simulink model "torque_vectoring_sim"  (R2022a)
settings: Solver=FixedStepAuto  StartTime=0.0  StopTime=5  FixedStep=0.01  RelTol=1e-3
undefined symbols (not defined in the file): DiscIntNeverNeededParam
libraries: simulink_extras x2, simulink x1
(part 1 of 2)
settings Model: Creator=mdrew  LastModifiedBy=mdrew

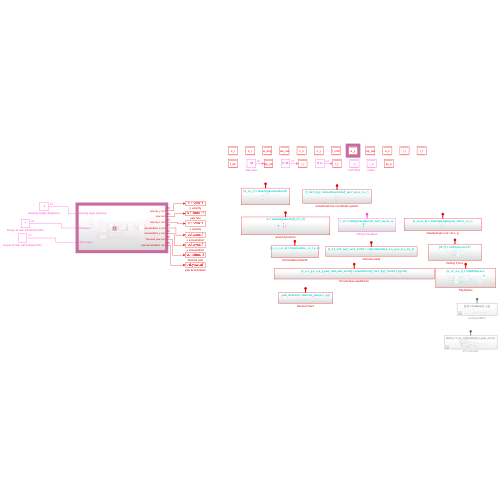
[thumbnail: Simulink's stored preview of the top-level diagram]
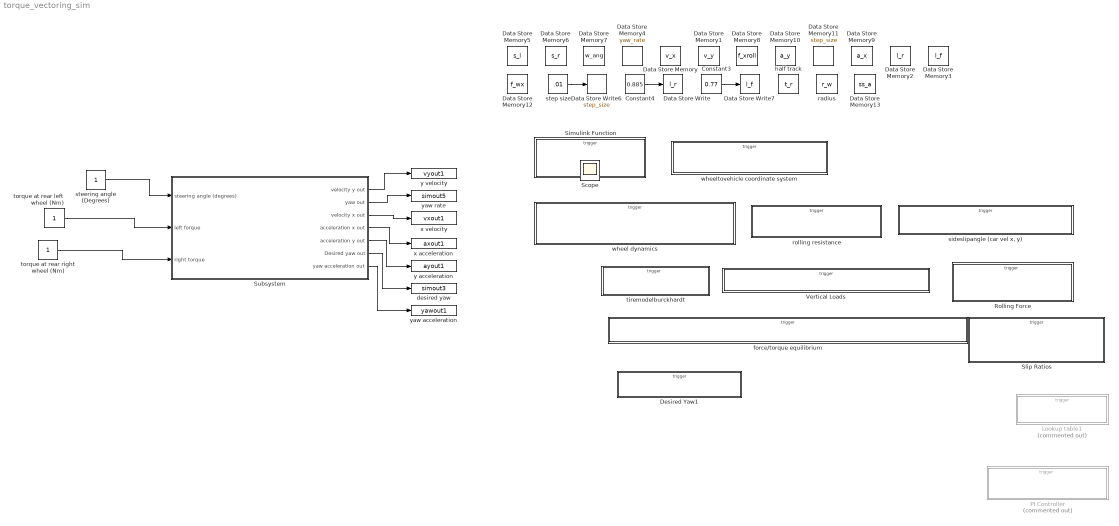
== system torque_vectoring_sim ==
  Constant3 : Constant  Value=0.77
  Constant4 : Constant  Value=0.885
  Data Store Memory : DataStoreMemory  DataStoreName=v_x  WriteAfterWriteMsg=warning  InitialValue=0.1  ShowAdditionalParam=off  OutMin=-10  OutMax=20
  Data Store Memory1 : DataStoreMemory  DataStoreName=v_y  WriteAfterWriteMsg=warning  InitialValue=0.0001  ShowAdditionalParam=off
  Data Store Memory10 : DataStoreMemory  DataStoreName=a_y  WriteAfterWriteMsg=warning  ShowAdditionalParam=off
  Data Store Memory11 : DataStoreMemory  DataStoreName=step_size  WriteAfterWriteMsg=warning  InitialValue=0.01  ShowAdditionalParam=off
  Data Store Memory12 : DataStoreMemory  DataStoreName=f_wx  WriteAfterWriteMsg=warning  InitialValue=[0.1, 0.1, 0.1, 0.1]  ShowAdditionalParam=off
  Data Store Memory13 : DataStoreMemory  DataStoreName=ss_a  WriteAfterWriteMsg=warning  InitialValue=[0, 0, 0, 0]  ShowAdditionalParam=off
  Data Store Memory2 : DataStoreMemory  DataStoreName=l_r  WriteAfterWriteMsg=warning  ShowAdditionalParam=off
  Data Store Memory3 : DataStoreMemory  DataStoreName=l_f  WriteAfterWriteMsg=warning  ShowAdditionalParam=off
  Data Store Memory4 : DataStoreMemory  DataStoreName=yaw_rate  WriteAfterWriteMsg=warning  InitialValue=0.001  ShowAdditionalParam=off
  Data Store Memory5 : DataStoreMemory  DataStoreName=s_l  WriteAfterWriteMsg=warning  ShowAdditionalParam=off
  Data Store Memory6 : DataStoreMemory  DataStoreName=s_r  WriteAfterWriteMsg=warning  ShowAdditionalParam=off
  Data Store Memory7 : DataStoreMemory  DataStoreName=w_ang  WriteAfterWriteMsg=warning  ShowAdditionalParam=off  Dimensions=4
  Data Store Memory8 : DataStoreMemory  DataStoreName=f_xroll  WriteAfterWriteMsg=warning  InitialValue=[.01, .01, .01, .01]  ShowAdditionalParam=off  Dimensions=4
  Data Store Memory9 : DataStoreMemory  DataStoreName=a_x  WriteAfterWriteMsg=warning  ShowAdditionalParam=off
  Data Store Write : DataStoreWrite  DataStoreName=l_r  IndexOptions=Index vector (dialog)  Indices=1  OutputSizes=1
  Data Store Write6 : DataStoreWrite  DataStoreName=step_size  IndexOptions=Index vector (dialog)  Indices=1  OutputSizes=1
  Data Store Write7 : DataStoreWrite  DataStoreName=l_f  IndexOptions=Index vector (dialog)  Indices=1  OutputSizes=1
  Desired Yaw1 : Subsystem  TreatAsAtomicUnit=on
  Lookup table1 : Subsystem  Commented=on  TreatAsAtomicUnit=on
  PI Controller : Subsystem  Commented=on  TreatAsAtomicUnit=on
  Rolling Force : Subsystem  TreatAsAtomicUnit=on
  Simulink Function : Subsystem  TreatAsAtomicUnit=on
  Slip Ratios : Subsystem  TreatAsAtomicUnit=on
  Subsystem : Subsystem
  Vertical Loads : Subsystem  TreatAsAtomicUnit=on
  desired yaw : ToWorkspace  VariableName=simout3  SaveFormat=Timeseries  SampleTime=-1
  force/torque equilibrium : Subsystem  TreatAsAtomicUnit=on
  half track : DataStoreMemory  DataStoreName=t_r  WriteAfterWriteMsg=warning  InitialValue=1.3208  ShowAdditionalParam=off
  radius : DataStoreMemory  DataStoreName=r_w  WriteAfterWriteMsg=warning  InitialValue=0.4572  ShowAdditionalParam=off
  rolling resistance : Subsystem  TreatAsAtomicUnit=on
  "sideslipangle (car vel x, y)" : Subsystem  TreatAsAtomicUnit=on
  steering angle (Degrees) : Constant
  step size : Constant  Value=.01
  tiremodelburckhardt : Subsystem  TreatAsAtomicUnit=on
  torque at rear left wheel (Nm) : Constant
  torque at rear right wheel (Nm) : Constant
  wheel dynamics : Subsystem  TreatAsAtomicUnit=on
  wheeltovehicle coordinate system : Subsystem  TreatAsAtomicUnit=on
  x acceleration : ToWorkspace  VariableName=axout1  SaveFormat=Timeseries  SampleTime=-1
  x velocity : ToWorkspace  VariableName=vxout1  SaveFormat=Timeseries  SampleTime=-1
  y acceleration : ToWorkspace  VariableName=ayout1  SaveFormat=Timeseries  SampleTime=-1
  y velocity : ToWorkspace  VariableName=vyout1  SaveFormat=Timeseries  SampleTime=-1
  yaw acceleration : ToWorkspace  VariableName=yawout1  SaveFormat=Timeseries  SampleTime=-1
  yaw rate : ToWorkspace  VariableName=simout5  SaveFormat=Timeseries  SampleTime=-1
  Scope : Scope
  wires:
  step size/1 -> Data Store Write6/1
  Constant4/1 -> Data Store Write/1
  Constant3/1 -> Data Store Write7/1
  torque at rear left wheel (Nm)/1 -> Subsystem/2(left forque)
  torque at rear right wheel (Nm)/1 -> Subsystem/3(right torque)
  steering angle (Degrees)/1 -> Subsystem/1(steering angle (degrees))
  Subsystem/6(Desired yaw out) -> desired yaw/1
  Subsystem/7(yaw acceleration out) -> yaw acceleration/1
  Subsystem/5(acceleration y out) -> y acceleration/1
  Subsystem/4(acceleration x out) -> x acceleration/1
  Subsystem/3(velocity x out) -> x velocity/1
  Subsystem/2(yaw out) -> yaw rate/1
  Subsystem/1(velocity y out) -> y velocity/1

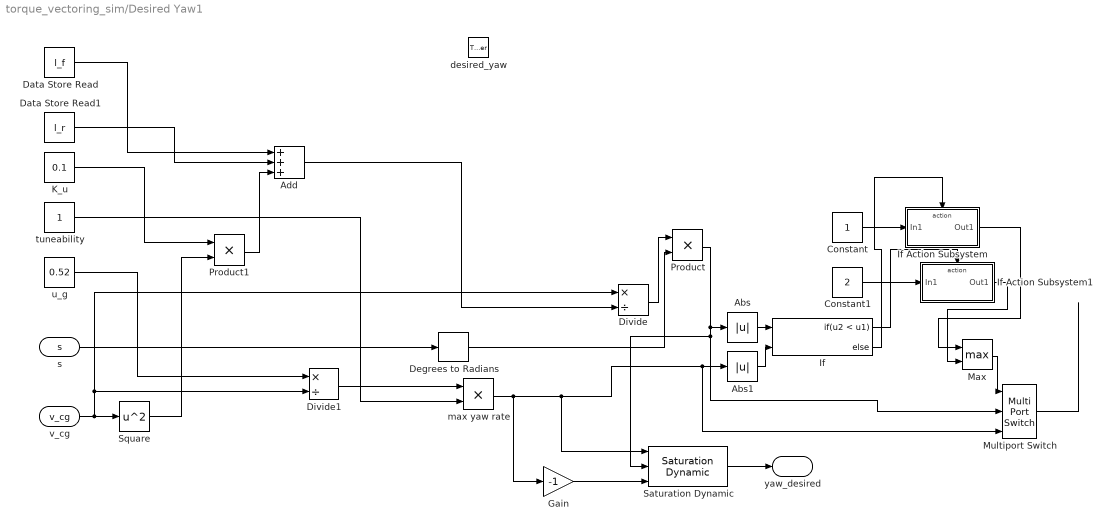
== system torque_vectoring_sim/Desired Yaw1 ==
  desired_yaw : TriggerPort  TriggerType=function-call  IsSimulinkFunction=on  FunctionName=desired_yaw  FunctionVisibility=scoped  VariantControl=(inherit)
  Abs : Abs  SaturateOnIntegerOverflow=off
  Abs1 : Abs  SaturateOnIntegerOverflow=off
  Add : Sum  Inputs=+++
  Constant : Constant
  Constant1 : Constant  Value=2
  Data Store Read : DataStoreRead  DataStoreName=l_f  IndexOptions=Index vector (dialog)  Indices=1  OutputSizes=1
  Data Store Read1 : DataStoreRead  DataStoreName=l_r  IndexOptions=Index vector (dialog)  Indices=1  OutputSizes=1
  Degrees to Radians : simulink_extras/Transformations/Degrees to Radians
  Divide : Product  Inputs=*/
  Divide1 : Product  Inputs=*/
  Gain : Gain  Gain=-1
  If : If  NumInputs=2  IfExpression=u2 < u1
  If Action Subsystem : Subsystem  TreatAsAtomicUnit=on
  If Action Subsystem1 : Subsystem  TreatAsAtomicUnit=on
  K_u : Constant  Value=0.1
  Max : MinMax  Function=max  Inputs=2
  Multiport Switch : MultiPortSwitch  Inputs=2  SaturateOnIntegerOverflow=off  InputSameDT=off
  Product : Product
  Product1 : Product
  Saturation Dynamic : simulink/Discontinuities/Saturation Dynamic  OutMin=[]  OutMax=[]  OutDataTypeStr=Inherit: Same as second input  OutDataType=fixdt(1, 16)  OutScaling=2^-10  DoSatur=off
  Square : Math  Operator=square
  max yaw rate : Product
  tuneability : Constant
  u_g : Constant  Value=0.52
  s : ArgIn  DisableCoverage=on  ArgumentName=s
  v_cg : ArgIn  Port=2  ArgumentName=v_cg
  yaw_desired : ArgOut  DisableCoverage=on  ArgumentName=yaw_desired
  wires:
  v_cg/1 -> Divide1/2, Divide/1, Square/1
  Divide/1 -> Product/1
  s/1 -> Degrees to Radians/1
  Data Store Read/1 -> Add/1
  Data Store Read1/1 -> Add/2
  Product1/1 -> Add/3
  K_u/1 -> Product1/1
  Square/1 -> Product1/2
  Add/1 -> Divide/2
  tuneability/1 -> max yaw rate/2
  Divide1/1 -> max yaw rate/1
  u_g/1 -> Divide1/1
  Product/1 -> Saturation Dynamic/2, Multiport Switch/2, Abs/1
  Abs/1 -> If/1
  Abs1/1 -> If/2
  max yaw rate/1 -> Gain/1, Saturation Dynamic/1, Multiport Switch/3, Abs1/1
  If Action Subsystem1/1(Out1) -> Max/2
  If/2 -> If Action Subsystem/Action
  Constant/1 -> If Action Subsystem/1(In1)
  Constant1/1 -> If Action Subsystem1/1(In1)
  If/1 -> If Action Subsystem1/Action
  If Action Subsystem/1(Out1) -> Max/1
  Max/1 -> Multiport Switch/1
  Multiport Switch/1 -> ?
  Degrees to Radians/1 -> Product/2
  Gain/1 -> Saturation Dynamic/3
  Saturation Dynamic/1 -> yaw_desired/1

== system torque_vectoring_sim/Lookup table1 ==
  lookup : TriggerPort  TriggerType=function-call  IsSimulinkFunction=on  FunctionName=lookup  FunctionVisibility=scoped  VariantControl=(inherit)
  i lookup Table1 : Lookup_n-D  NumberOfTableDimensions=1  BreakpointsForDimension1=[7 10 13 16 19 22]  Table=[12716.7 12492.5 12040 11536.07 11058.5 13650]  InternalRulePriority=Speed  RndMeth=Simplest
  p lookup Table : Lookup_n-D  NumberOfTableDimensions=1  BreakpointsForDimension1=[7 10 13 16 19 22]  Table=[296.29 392.23 421.72 479.87 396.22 404.79]  InternalRulePriority=Speed  RndMeth=Simplest
  v_cg : ArgIn  DisableCoverage=on  ArgumentName=v_cg
  p : ArgOut  DisableCoverage=on  ArgumentName=p
  i : ArgOut  Port=2  ArgumentName=i
  wires:
  v_cg/1 -> i lookup Table1/1, p lookup Table/1
  i lookup Table1/1 -> i/1
  p lookup Table/1 -> p/1

== system torque_vectoring_sim/PI Controller ==
  pi_controller : TriggerPort  TriggerType=function-call  IsSimulinkFunction=on  FunctionName=pi_controller  FunctionVisibility=scoped  VariantControl=(inherit)
  Add : Sum
  Constant : Constant
  Discrete-Time Integrator : DiscreteIntegrator  SampleTime=-1  ICPrevOutput=DiscIntNeverNeededParam  ICPrevScaledInput=DiscIntNeverNeededParam
  Divide : Product  Inputs=*/
  Divide1 : Product  Inputs=*/
  Product{,1..3} (4 alike) : Product
  Sum : Sum  Inputs=|++
  delta torque out : ToWorkspace  VariableName=simout2  SaveFormat=Timeseries  SampleTime=-1
  p : ArgIn  DisableCoverage=on  ArgumentName=p
  i : ArgIn  Port=2  ArgumentName=i
  yaw_error : ArgIn  Port=3  ArgumentName=yaw_error
  delta_t : ArgOut  DisableCoverage=on  ArgumentName=delta_t
  wires:
  p/1 -> Product2/2, Divide/1, Product1/1
  i/1 -> Divide/2, Product/1
  Sum/1 -> ?
  yaw_error/1 -> Product3/2, Product1/2, Discrete-Time Integrator/1
  Discrete-Time Integrator/1 -> Product/2
  Product/1 -> Sum/2
  Product1/1 -> Sum/1
  Constant/1 -> Add/1, Divide1/1
  Divide/1 -> Product3/1
  Divide1/1 -> Add/2
  Add/1 -> Product2/1
  Product2/1 -> delta torque out/1, delta_t/1
  Product3/1 -> Divide1/2

== system torque_vectoring_sim/Rolling Force ==
  rolFor : TriggerPort  TriggerType=function-call  IsSimulinkFunction=on  FunctionName=rolFor  FunctionVisibility=scoped  VariantControl=(inherit)
  Asphalt Road Condition (c_roll) : Constant  Value=0.01
  Concrete Road Condition (c_roll) : Constant  Value=0.008
  F_xroll : MATLAB Function  TreatAsAtomicUnit=on
  F_yroll : MATLAB Function  TreatAsAtomicUnit=on
  Vector Concatenate1 : Concatenate
  Vector Concatenate2 : Concatenate  NumInputs=4
  w : ArgIn  DisableCoverage=on  PortDimensions=4  ArgumentName=w
  sl : ArgIn  DisableCoverage=on  Port=2  ArgumentName=sl
  sr : ArgIn  DisableCoverage=on  Port=3  ArgumentName=sr
  F : ArgIn  Port=4  PortDimensions=4  ArgumentName=F
  X : ArgOut  DisableCoverage=on  PortDimensions=4  ArgumentName=X
  Y : ArgOut  DisableCoverage=on  Port=2  PortDimensions=2  ArgumentName=Y
  wires:
  Asphalt Road Condition (c_roll)/1 -> F_yroll/1(c), F_xroll/1(c)
  F/1 -> F_yroll/2(f), F_xroll/2(f)
  w/1 -> F_yroll/3(w), F_xroll/3(w)
  sl/1 -> F_yroll/4(sl), F_xroll/4(sl)
  Vector Concatenate2/1 -> X/1
  Vector Concatenate1/1 -> Y/1
  F_yroll/2(fr) -> Vector Concatenate1/2
  F_yroll/1(fl) -> Vector Concatenate1/1
  F_xroll/3(rl) -> Vector Concatenate2/3
  F_xroll/2(fr) -> Vector Concatenate2/2
  F_xroll/1(fl) -> Vector Concatenate2/1
  F_xroll/4(rr) -> Vector Concatenate2/4
  sr/1 -> F_xroll/5(sr), F_yroll/5(sr)

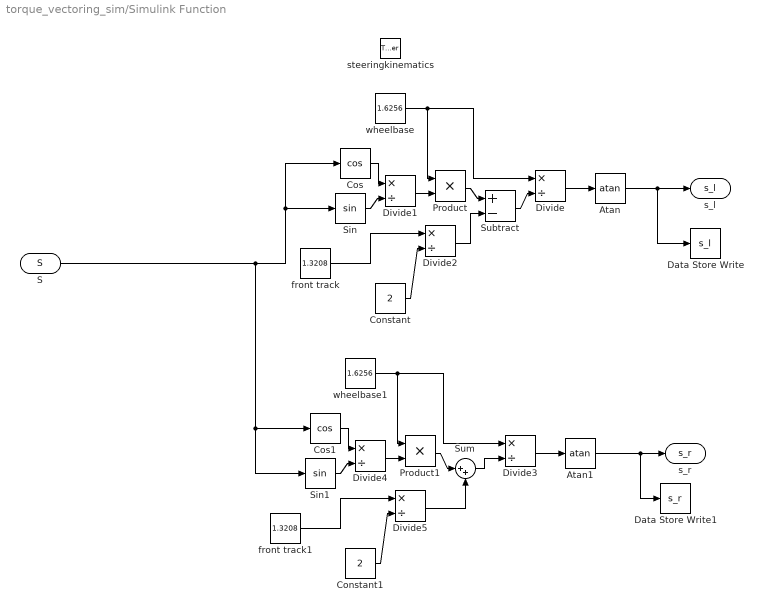
== system torque_vectoring_sim/Simulink Function ==
  steeringkinematics : TriggerPort  TriggerType=function-call  IsSimulinkFunction=on  FunctionName=steeringkinematics  FunctionVisibility=scoped  VariantControl=(inherit)
  Atan : Trigonometry  Operator=atan
  Atan1 : Trigonometry  Operator=atan
  Constant : Constant  Value=2
  Constant1 : Constant  Value=2
  Cos : Trigonometry  Operator=cos
  Cos1 : Trigonometry  Operator=cos
  Data Store Write : DataStoreWrite  DataStoreName=s_l  IndexOptions=Index vector (dialog)  Indices=1  OutputSizes=1
  Data Store Write1 : DataStoreWrite  DataStoreName=s_r  IndexOptions=Index vector (dialog)  Indices=1  OutputSizes=1
  Divide{,1..5} (6 alike) : Product  Inputs=*/
  Product : Product
  Product1 : Product
  Sin : Trigonometry
  Sin1 : Trigonometry
  Subtract : Sum  Inputs=+-
  Sum : Sum  Inputs=|++
  front track : Constant  Value=1.3208
  front track1 : Constant  Value=1.3208
  wheelbase : Constant  Value=1.6256
  wheelbase1 : Constant  Value=1.6256
  S : ArgIn  DisableCoverage=on  ArgumentName=S
  s_l : ArgOut  DisableCoverage=on  ArgumentName=s_l
  s_r : ArgOut  DisableCoverage=on  Port=2  ArgumentName=s_r
  wires:
  Divide/1 -> Atan/1
  Divide1/1 -> Product/2
  Product/1 -> Subtract/1
  Divide2/1 -> Subtract/2
  Atan/1 -> Data Store Write/1, s_l/1
  wheelbase/1 -> Product/1, Divide/1
  Subtract/1 -> Divide/2
  Sin/1 -> Divide1/2
  Cos/1 -> Divide1/1
  Constant/1 -> Divide2/2
  front track/1 -> Divide2/1
  S/1 -> Sin1/1, Cos1/1, Cos/1, Sin/1
  wheelbase1/1 -> Product1/1, Divide3/1
  Divide5/1 -> Sum/2
  Constant1/1 -> Divide5/2
  front track1/1 -> Divide5/1
  Product1/1 -> Sum/1
  Sin1/1 -> Divide4/2
  Divide4/1 -> Product1/2
  Sum/1 -> Divide3/2
  Cos1/1 -> Divide4/1
  Divide3/1 -> Atan1/1
  Atan1/1 -> Data Store Write1/1, s_r/1

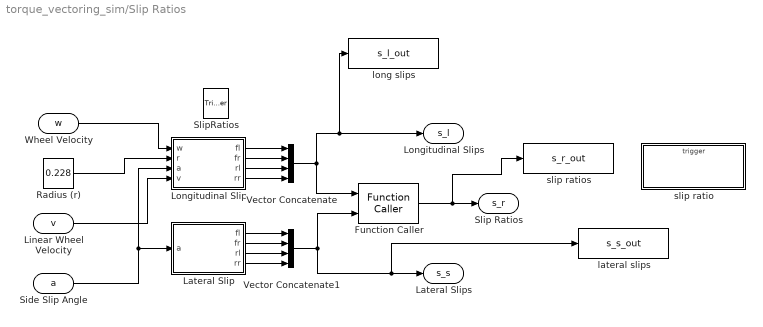
== system torque_vectoring_sim/Slip Ratios ==
  SlipRatios : TriggerPort  TriggerType=function-call  IsSimulinkFunction=on  FunctionName=slipRat  FunctionVisibility=scoped  VariantControl=(inherit)
  Function Caller : FunctionCaller  FunctionPrototype=sr = slipratio(sl,ss)  InputArgumentSpecifications=<Enter example>  OutputArgumentSpecifications=<Enter example>
  Lateral Slip : MATLAB Function  TreatAsAtomicUnit=on
  Longitudinal Slip : MATLAB Function  TreatAsAtomicUnit=on
  Radius (r) : Constant  Value=0.228
  Vector Concatenate : Concatenate  NumInputs=4
  Vector Concatenate1 : Concatenate  NumInputs=4
  lateral slips : ToWorkspace  VariableName=s_s_out  SaveFormat=Timeseries  SampleTime=-1
  long slips : ToWorkspace  VariableName=s_l_out  SaveFormat=Timeseries  SampleTime=-1
  slip ratio : Subsystem  TreatAsAtomicUnit=on
  slip ratios : ToWorkspace  VariableName=s_r_out  SaveFormat=Timeseries  SampleTime=-1
  Wheel Velocity : ArgIn  DisableCoverage=on  PortDimensions=4  ArgumentName=w
  Side Slip Angle : ArgIn  DisableCoverage=on  Port=2  PortDimensions=4  ArgumentName=a
  Linear Wheel Velocity : ArgIn  DisableCoverage=on  Port=3  PortDimensions=4  ArgumentName=v
  Longitudinal Slips : ArgOut  DisableCoverage=on  PortDimensions=4  ArgumentName=s_l
  Lateral Slips : ArgOut  DisableCoverage=on  Port=2  PortDimensions=4  ArgumentName=s_s
  Slip Ratios : ArgOut  DisableCoverage=on  Port=3  PortDimensions=4  ArgumentName=s_r
  wires:
  Side Slip Angle/1 -> Longitudinal Slip/3(a), Lateral Slip/1(a)
  Vector Concatenate/1 -> Function Caller/1, long slips/1, Longitudinal Slips/1
  Vector Concatenate1/1 -> Function Caller/2, lateral slips/1, Lateral Slips/1
  Longitudinal Slip/1(fl) -> Vector Concatenate/1
  Longitudinal Slip/2(fr) -> Vector Concatenate/2
  Longitudinal Slip/3(rl) -> Vector Concatenate/3
  Longitudinal Slip/4(rr) -> Vector Concatenate/4
  Lateral Slip/1(fl) -> Vector Concatenate1/1
  Lateral Slip/2(fr) -> Vector Concatenate1/2
  Lateral Slip/3(rl) -> Vector Concatenate1/3
  Lateral Slip/4(rr) -> Vector Concatenate1/4
  Linear Wheel Velocity/1 -> Longitudinal Slip/4(v)
  Radius (r)/1 -> Longitudinal Slip/2(r)
  Function Caller/1 -> slip ratios/1, Slip Ratios/1
  Wheel Velocity/1 -> Longitudinal Slip/1(w)

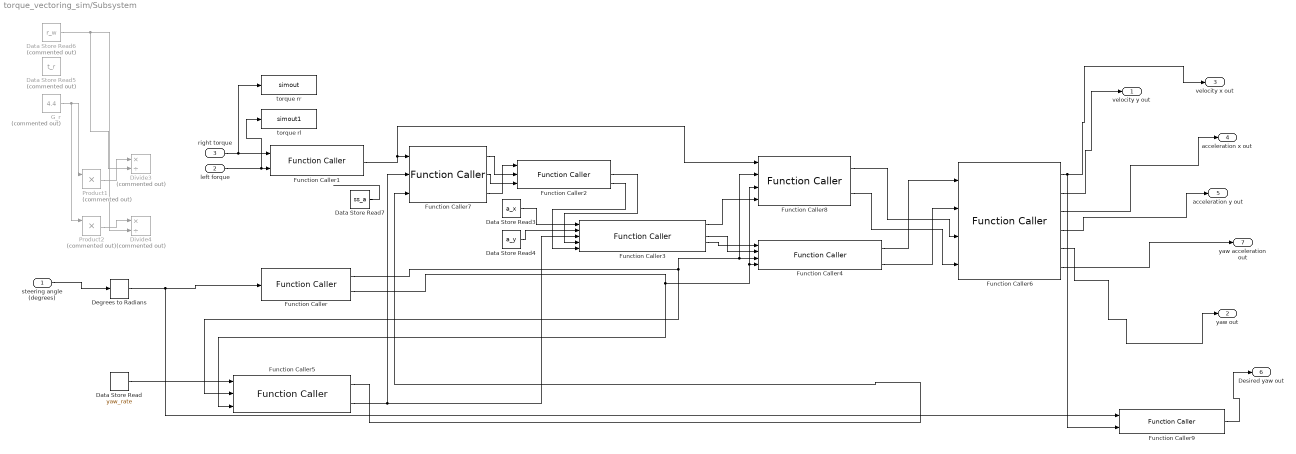
== system torque_vectoring_sim/Subsystem ==
  steering angle (degrees) : Inport
  left forque : Inport  Port=2
  right torque : Inport  Port=3
  Data Store Read : DataStoreRead  DataStoreName=yaw_rate  IndexOptions=Index vector (dialog)  Indices=1  OutputSizes=1
  Data Store Read3 : DataStoreRead  DataStoreName=a_x  IndexOptions=Index vector (dialog)  Indices=1  OutputSizes=1
  Data Store Read4 : DataStoreRead  DataStoreName=a_y  IndexOptions=Index vector (dialog)  Indices=1  OutputSizes=1
  Data Store Read5 : DataStoreRead  Commented=on  DataStoreName=t_r  IndexOptions=Index vector (dialog)  Indices=1  OutputSizes=1
  Data Store Read6 : DataStoreRead  Commented=on  DataStoreName=r_w  IndexOptions=Index vector (dialog)  Indices=1  OutputSizes=1
  Data Store Read7 : DataStoreRead  DataStoreName=ss_a  IndexOptions=Index vector (dialog)  Indices=1  OutputSizes=1
  Degrees to Radians : simulink_extras/Transformations/Degrees to Radians
  Divide3 : Product  Commented=on  Inputs=*/
  Divide4 : Product  Commented=on  Inputs=*/
  Function Caller : FunctionCaller  FunctionPrototype=[s_l,s_r] = steeringkinematics(S)  InputArgumentSpecifications=<Enter example>  OutputArgumentSpecifications=<Enter example>
  Function Caller1 : FunctionCaller  FunctionPrototype=w = wheeldynamics(t_rr,t_rl)  InputArgumentSpecifications=<Enter example>  OutputArgumentSpecifications=<Enter example>
  Function Caller2 : FunctionCaller  FunctionPrototype=[u_r,u_l,u_s] = tiremodel(s_r,s_l,s_s)  InputArgumentSpecifications=<Enter example>  OutputArgumentSpecifications=<Enter example>
  Function Caller3 : FunctionCaller  FunctionPrototype=[f_z,f_wl,f_wy,f_wx,f_xroll] = verticalloads(a_x,a_y,ss_a,u_l,u_s)  InputArgumentSpecifications=<Enter example>  OutputArgumentSpecifications=<Enter example>
  Function Caller4 : FunctionCaller  FunctionPrototype=[f_bx,f_by] = wheeltovehicle(f_wx,f_wy,s_l,s_r)  OutputArgumentSpecifications=<Enter example>
  Function Caller5 : FunctionCaller  FunctionPrototype=[v_w,ss_a] = sideslipangle(yaw_rate,s_l,s_r)  InputArgumentSpecifications=<Enter example>  OutputArgumentSpecifications=<Enter example>
  Function Caller6 : FunctionCaller  FunctionPrototype=[v_x,v_y,a_x,a_y,yaw_rate,yaw_accel] = equilibrium(f_bx,f_by,f_bxroll,f_byroll)  InputArgumentSpecifications=<Enter example>  OutputArgumentSpecifications=<Enter example>
  Function Caller7 : FunctionCaller  FunctionPrototype=[s_l,s_s,s_r] = slipRat(w,a,v)  InputArgumentSpecifications=<Enter example>  OutputArgumentSpecifications=<Enter example>
  Function Caller8 : FunctionCaller  FunctionPrototype=[X,Y] = rolFor(w,sl,sr,F)  InputArgumentSpecifications=<Enter example>  OutputArgumentSpecifications=<Enter example>
  Function Caller9 : FunctionCaller  FunctionPrototype=yaw_desired = desired_yaw(s,v_cg)  InputArgumentSpecifications=<Enter example>  OutputArgumentSpecifications=<Enter example>
  G_r : Constant  Commented=on  Value=4.4
  Product1 : Product  Commented=on
  Product2 : Product  Commented=on
  torque rl : ToWorkspace  VariableName=simout1  SaveFormat=Timeseries  SampleTime=-1
  torque rr : ToWorkspace  VariableName=simout  SaveFormat=Timeseries  SampleTime=-1
  velocity y out : Outport
  yaw out : Outport  Port=2
  velocity x out : Outport  Port=3
  acceleration x out : Outport  Port=4
  acceleration y out : Outport  Port=5
  Desired yaw out : Outport  Port=6
  yaw acceleration out : Outport  Port=7
  wires:
  Function Caller/1 -> Function Caller5/2, Function Caller8/2, Function Caller4/3
  Function Caller3/1 -> Function Caller8/4
  Function Caller7/2 -> Function Caller2/3
  Data Store Read3/1 -> Function Caller3/1
  Data Store Read4/1 -> Function Caller3/2
  Function Caller5/1 -> Function Caller7/3
  Function Caller3/3 -> Function Caller4/2
  Function Caller/2 -> Function Caller8/3, Function Caller4/4, Function Caller5/3
  Function Caller8/2 -> Function Caller6/4
  Function Caller6/5 -> yaw out/1
  Degrees to Radians/1 -> Function Caller9/1, Function Caller/1
  Function Caller6/2 -> velocity y out/1
  Function Caller6/3 -> acceleration x out/1
  Function Caller6/4 -> acceleration y out/1
  Function Caller2/2 -> Function Caller3/4
  Function Caller7/3 -> Function Caller2/1
  Function Caller3/4 -> Function Caller4/1
  Function Caller4/1 -> Function Caller6/1
  Function Caller4/2 -> Function Caller6/2
  Function Caller1/1 -> Function Caller8/1, Function Caller7/1
  Function Caller7/1 -> Function Caller2/2
  Function Caller8/1 -> Function Caller6/3
  Function Caller2/3 -> Function Caller3/5
  steering angle (degrees)/1 -> Degrees to Radians/1
  G_r/1 -> Product2/1, Product1/1
  Data Store Read6/1 -> Divide3/2, Divide4/2
  Data Store Read/1 -> Function Caller5/1
  left forque/1 -> torque rl/1, Function Caller1/2
  Product1/1 -> Divide3/1
  Product2/1 -> Divide4/1
  Function Caller6/6 -> yaw acceleration out/1
  Data Store Read7/1 -> ?
  Function Caller5/2 -> Function Caller3/3, Function Caller7/2
  Function Caller9/1 -> Desired yaw out/1
  right torque/1 -> torque rr/1, Function Caller1/1
  Function Caller6/1 -> Function Caller9/2, velocity x out/1

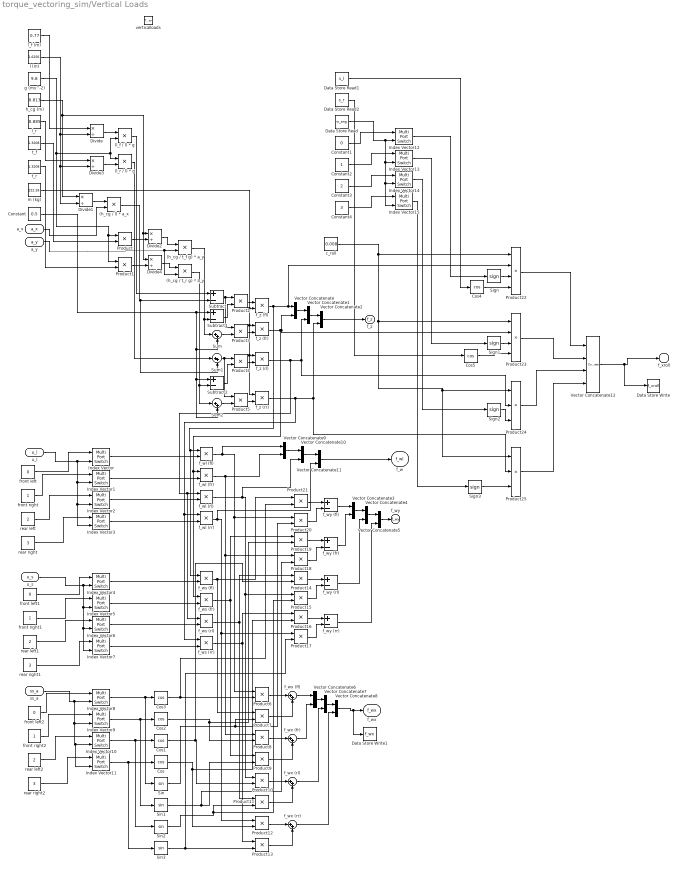
== system torque_vectoring_sim/Vertical Loads ==
  verticalloads : TriggerPort  TriggerType=function-call  IsSimulinkFunction=on  FunctionName=verticalloads  FunctionVisibility=scoped  VariantControl=(inherit)
  (h_cg / l) * a_x : Product
  (h_cg / t_f g) * a_y : Product
  (h_cg / t_r g) * a_y : Product
  (l_f / l) * g : Product
  (l_r / l) * g : Product
  Constant : Constant  Value=0.5
  Constant1 : Constant  Value=0
  Constant2 : Constant
  Constant3 : Constant  Value=2
  Constant4 : Constant  Value=3
  Cos{,1..5} (6 alike) : Trigonometry  Operator=cos
  Data Store Read : DataStoreRead  DataStoreName=w_ang  IndexOptions=Index vector (dialog)  Indices=1  OutputSizes=1
  Data Store Read1 : DataStoreRead  DataStoreName=s_l  IndexOptions=Index vector (dialog)  Indices=1  OutputSizes=1
  Data Store Read2 : DataStoreRead  DataStoreName=s_r  IndexOptions=Index vector (dialog)  Indices=1  OutputSizes=1
  Data Store Write : DataStoreWrite  DataStoreName=f_xroll  IndexOptions=Index vector (dialog)  Indices=1  OutputSizes=1
  Data Store Write1 : DataStoreWrite  DataStoreName=f_wx  IndexOptions=Index vector (dialog)  Indices=1  OutputSizes=1
  Divide{,1..4} (5 alike) : Product  Inputs=*/
  Index Vector{,1..15} (16 alike) : MultiPortSwitch  DataPortOrder=Zero-based contiguous  Inputs=1  zeroidx=on  SaturateOnIntegerOverflow=off  InputSameDT=off
  Product{,1..21} (22 alike) : Product
  Product22 : Product  Inputs=4
  Product23 : Product  Inputs=4
  Product24 : Product  Inputs=3
  Product25 : Product  Inputs=3
  Sign{,1..3} (4 alike) : Signum
  Sin{,1..3} (4 alike) : Trigonometry
  Subtract : Sum  Inputs=+-
  Subtract1 : Sum  Inputs=+-
  Subtract2 : Sum  Inputs=+-
  Sum : Sum  Inputs=|++
  Sum1 : Sum  Inputs=|++
  Sum2 : Sum  Inputs=|++
  Vector Concatenate{,1..11} (12 alike) : Concatenate
  Vector Concatenate12 : Concatenate  NumInputs=4
  c_roll : Constant  Value=0.008
  f_wl (fl) : Product
  f_wl (fr) : Product
  f_wl (rl) : Product
  f_wl (rr) : Product
  f_ws (fl) : Product
  f_ws (fr) : Product
  f_ws (rl) : Product
  f_ws (rr) : Product
  f_wx (fl) : Sum  Inputs=|++
  f_wx (fr) : Sum  Inputs=|++
  f_wx (rl) : Sum  Inputs=|++
  f_wx (rr) : Sum  Inputs=|++
  f_wy (fl) : Sum  Inputs=+-
  f_wy (fr) : Sum  Inputs=+-
  f_wy (rl) : Sum  Inputs=+-
  f_wy (rr) : Sum  Inputs=+-
  f_z (fl) : Product
  f_z (fr) : Product
  f_z (rl) : Product
  f_z (rr) : Product
  front left : Constant  Value=0
  front left1 : Constant  Value=0
  front left2 : Constant  Value=0
  front right : Constant
  front right1 : Constant
  front right2 : Constant
  g (ms^-2) : Constant  Value=9.8
  h_cg (m) : Constant  Value=0.813
  l (m) : Constant  Value=1.6256
  l_f (m) : Constant  Value=0.77
  l_r : Constant  Value=0.885
  m (kg) : Constant  Value=222.26
  rear left : Constant  Value=2
  rear left1 : Constant  Value=2
  rear left2 : Constant  Value=2
  rear right : Constant  Value=3
  rear right1 : Constant  Value=3
  rear right2 : Constant  Value=3
  t_f : Constant  Value=1.3208
  t_r : Constant  Value=1.3208
  a_x : ArgIn  ArgumentName=a_x
  a_y : ArgIn  Port=2  ArgumentName=a_y
  ss_a : ArgIn  Port=3  PortDimensions=4  ArgumentName=ss_a
  u_l : ArgIn  Port=4  PortDimensions=4  ArgumentName=u_l
  u_s : ArgIn  Port=5  PortDimensions=4  ArgumentName=u_s
  f_z : ArgOut  PortDimensions=4  ArgumentName=f_z
  f_w : ArgOut  Port=2  PortDimensions=4  ArgumentName=f_wl
  f_wy : ArgOut  Port=3  PortDimensions=4  ArgumentName=f_wy
  f_wx : ArgOut  Port=4  PortDimensions=4  ArgumentName=f_wx
  f_xroll : ArgOut  Port=5  PortDimensions=4  ArgumentName=f_xroll
  wires:
  l_f (m)/1 -> Divide/1
  l (m)/1 -> Divide3/2, Divide1/2, Divide/2
  Divide/1 -> (l_f / l) * g/1
  g (ms^-2)/1 -> Product1/1, Product/1, (l_r / l) * g/1, (l_f / l) * g/2
  Divide1/1 -> (h_cg / l) * a_x/1
  a_x/1 -> (h_cg / l) * a_x/2
  h_cg (m)/1 -> Divide2/1, Divide4/1, Divide1/1
  Product/1 -> Divide2/2
  t_f/1 -> Product/2
  Divide2/1 -> (h_cg / t_f g) * a_y/1
  a_y/1 -> (h_cg / t_r g) * a_y/2, (h_cg / t_f g) * a_y/2
  l_r/1 -> Divide3/1
  Divide3/1 -> (l_r / l) * g/2
  t_r/1 -> Product1/2
  Product1/1 -> Divide4/2
  Divide4/1 -> (h_cg / t_r g) * a_y/1
  (l_f / l) * g/1 -> Subtract/1
  (h_cg / l) * a_x/1 -> Sum1/2, Subtract/2
  (h_cg / t_f g) * a_y/1 -> Sum/1, Subtract1/2
  Subtract/1 -> Product3/1, Product2/1
  Subtract1/1 -> Product2/2
  Product2/1 -> f_z (fl)/1
  m (kg)/1 -> f_z (rr)/1, f_z (rl)/1, f_z (fr)/1, f_z (fl)/2
  Constant/1 -> Sum2/2, Subtract2/1, Sum/2, Subtract1/1
  Sum/1 -> Product3/2
  Product3/1 -> f_z (fr)/2
  (l_r / l) * g/1 -> Sum1/1
  (h_cg / t_r g) * a_y/1 -> Sum2/1, Subtract2/2
  Sum1/1 -> Product5/1, Product4/1
  Subtract2/1 -> Product4/2
  Product4/1 -> f_z (rl)/2
  Sum2/1 -> Product5/2
  Product5/1 -> f_z (rr)/2
  f_z (fr)/1 -> f_ws (fr)/1, f_wl (fr)/1, Vector Concatenate/2, Product23/2
  Vector Concatenate/1 -> Vector Concatenate1/1
  f_z (rl)/1 -> f_ws (rl)/1, f_wl (rl)/1, Product24/2, Vector Concatenate1/2
  Vector Concatenate1/1 -> Vector Concatenate2/1
  f_z (rr)/1 -> f_ws (rr)/1, f_wl (rr)/1, Vector Concatenate2/2, Product25/2
  Vector Concatenate2/1 -> f_z/1
  Index Vector/1 -> f_wl (fl)/2
  f_z (fl)/1 -> f_ws (fl)/1, f_wl (fl)/1, Product22/2, Vector Concatenate/1
  Index Vector1/1 -> f_wl (fr)/2
  Index Vector2/1 -> f_wl (rl)/2
  Index Vector3/1 -> f_wl (rr)/2
  Index Vector4/1 -> f_ws (fl)/2
  Index Vector5/1 -> f_ws (fr)/2
  Index Vector6/1 -> f_ws (rl)/2
  Index Vector7/1 -> f_ws (rr)/2
  Product6/1 -> f_wx (fl)/1
  Product7/1 -> f_wx (fl)/2
  Product9/1 -> f_wx (fr)/2
  Product8/1 -> f_wx (fr)/1
  Product11/1 -> f_wx (rl)/2
  Product10/1 -> f_wx (rl)/1
  Product13/1 -> f_wx (rr)/2
  Product12/1 -> f_wx (rr)/1
  Index Vector8/1 -> Sin/1, Cos3/1
  Index Vector11/1 -> Sin3/1, Cos/1
  Index Vector9/1 -> Sin1/1, Cos2/1
  f_wl (fl)/1 -> Vector Concatenate9/1, Product20/1, Product6/1
  Cos/1 -> Product12/2, Product16/2
  f_wl (fr)/1 -> Vector Concatenate9/2, Product18/1, Product8/1
  f_wl (rl)/1 -> Vector Concatenate10/2, Product15/1, Product10/1
  f_wl (rr)/1 -> Vector Concatenate11/2, Product17/1, Product12/1
  f_ws (fl)/1 -> Product21/1, Product7/1
  f_ws (fr)/1 -> Product9/1, Product19/1
  f_ws (rl)/1 -> Product11/1, Product14/1
  f_ws (rr)/1 -> Product13/1, Product16/1
  Index Vector10/1 -> Sin2/1, Cos1/1
  Sin2/1 -> Product15/2, Product11/2
  Sin3/1 -> Product17/2, Product13/2
  Product21/1 -> f_wy (fl)/1
  Product20/1 -> f_wy (fl)/2
  Product16/1 -> f_wy (rr)/1
  Product17/1 -> f_wy (rr)/2
  Product14/1 -> f_wy (rl)/1
  Product15/1 -> f_wy (rl)/2
  Product18/1 -> f_wy (fr)/2
  Product19/1 -> f_wy (fr)/1
  Cos3/1 -> Product21/2, Product6/2
  Sin/1 -> Product20/2, Product7/2
  Cos2/1 -> Product19/2, Product8/2
  Sin1/1 -> Product18/2, Product9/2
  Cos1/1 -> Product14/2, Product10/2
  f_wy (fl)/1 -> Vector Concatenate3/1
  f_wy (fr)/1 -> Vector Concatenate3/2
  Vector Concatenate3/1 -> Vector Concatenate4/1
  f_wy (rl)/1 -> Vector Concatenate4/2
  Vector Concatenate4/1 -> Vector Concatenate5/1
  f_wy (rr)/1 -> Vector Concatenate5/2
  Vector Concatenate5/1 -> f_wy/1
  f_wx (fl)/1 -> Vector Concatenate6/1
  f_wx (fr)/1 -> Vector Concatenate6/2
  Vector Concatenate6/1 -> Vector Concatenate7/1
  f_wx (rl)/1 -> Vector Concatenate7/2
  Vector Concatenate7/1 -> Vector Concatenate8/1
  f_wx (rr)/1 -> Vector Concatenate8/2
  Vector Concatenate8/1 -> Data Store Write1/1, f_wx/1
  Vector Concatenate10/1 -> Vector Concatenate11/1
  Vector Concatenate9/1 -> Vector Concatenate10/1
  Vector Concatenate11/1 -> f_w/1
  rear right2/1 -> Index Vector11/1
  rear left2/1 -> Index Vector10/1
  front right2/1 -> Index Vector9/1
  front left2/1 -> Index Vector8/1
  ss_a/1 -> Index Vector11/2, Index Vector10/2, Index Vector9/2, Index Vector8/2
  u_s/1 -> Index Vector7/2, Index Vector6/2, Index Vector5/2, Index Vector4/2
  front left1/1 -> Index Vector4/1
  front right1/1 -> Index Vector5/1
  rear left1/1 -> Index Vector6/1
  rear right1/1 -> Index Vector7/1
  rear right/1 -> Index Vector3/1
  rear left/1 -> Index Vector2/1
  front right/1 -> Index Vector1/1
  front left/1 -> Index Vector/1
  u_l/1 -> Index Vector3/2, Index Vector2/2, Index Vector1/2, Index Vector/2
  c_roll/1 -> Product25/1, Product24/1, Product23/1, Product22/1
  Sign/1 -> Product22/3
  Sign1/1 -> Product23/3
  Sign2/1 -> Product24/3
  Sign3/1 -> Product25/3
  Constant1/1 -> Index Vector12/1
  Constant2/1 -> Index Vector13/1
  Constant3/1 -> Index Vector14/1
  Constant4/1 -> Index Vector15/1
  Data Store Read/1 -> Index Vector15/2, Index Vector14/2, Index Vector13/2, Index Vector12/2
  Index Vector12/1 -> Sign/1
  Cos4/1 -> Product22/4
  Data Store Read1/1 -> Cos4/1
  Cos5/1 -> Product23/4
  Data Store Read2/1 -> Cos5/1
  Index Vector13/1 -> Sign1/1
  Index Vector14/1 -> Sign2/1
  Index Vector15/1 -> Sign3/1
  Vector Concatenate12/1 -> Data Store Write/1, f_xroll/1
  Product25/1 -> Vector Concatenate12/4
  Product24/1 -> Vector Concatenate12/3
  Product23/1 -> Vector Concatenate12/2
  Product22/1 -> Vector Concatenate12/1

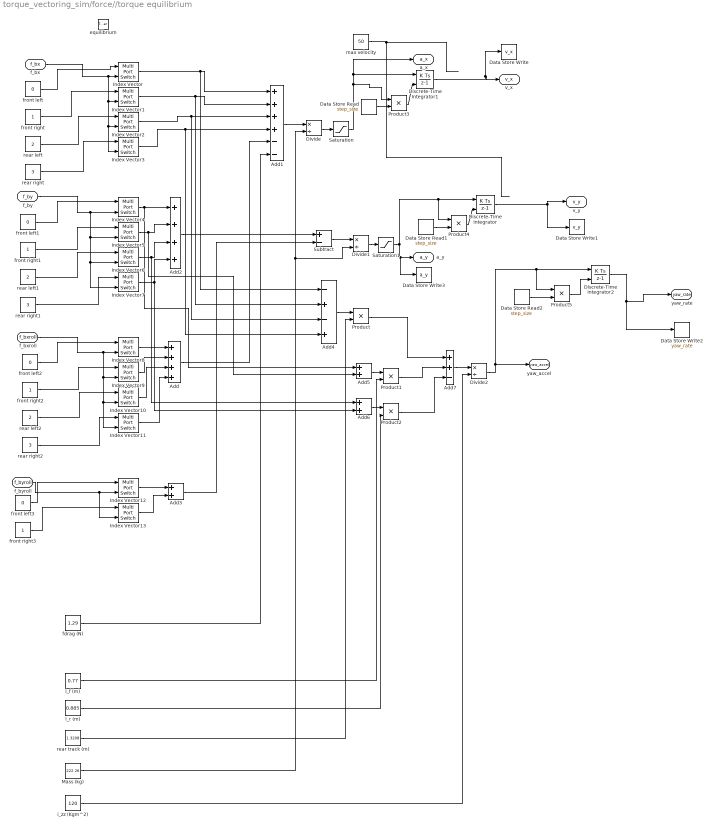
== system torque_vectoring_sim/force//torque equilibrium ==
  equilibrium : TriggerPort  TriggerType=function-call  IsSimulinkFunction=on  FunctionName=equilibrium  FunctionVisibility=scoped  VariantControl=(inherit)
  Add : Sum  Inputs=++++
  Add1 : Sum  Inputs=++++--
  Add2 : Sum  Inputs=++++
  Add3 : Sum
  Add4 : Sum  Inputs=-+-+
  Add5 : Sum
  Add6 : Sum
  Add7 : Sum  Inputs=++-
  Data Store Read : DataStoreRead  DataStoreName=step_size  IndexOptions=Index vector (dialog)  Indices=1  OutputSizes=1
  Data Store Read1 : DataStoreRead  DataStoreName=step_size  IndexOptions=Index vector (dialog)  Indices=1  OutputSizes=1
  Data Store Read2 : DataStoreRead  DataStoreName=step_size  IndexOptions=Index vector (dialog)  Indices=1  OutputSizes=1
  Data Store Write : DataStoreWrite  DataStoreName=v_x  IndexOptions=Index vector (dialog)  Indices=1  OutputSizes=1
  Data Store Write1 : DataStoreWrite  DataStoreName=v_y  IndexOptions=Index vector (dialog)  Indices=1  OutputSizes=1
  Data Store Write2 : DataStoreWrite  DataStoreName=yaw_rate  IndexOptions=Index vector (dialog)  Indices=1  OutputSizes=1
  Data Store Write3 : DataStoreWrite  DataStoreName=a_y  IndexOptions=Index vector (dialog)  Indices=1  OutputSizes=1
  Discrete-Time Integrator : DiscreteIntegrator  InitialConditionSource=external  SampleTime=-1  LimitOutput=on  UpperSaturationLimit=50  LowerSaturationLimit=-50  ICPrevOutput=DiscIntNeverNeededParam  ICPrevScaledInput=DiscIntNeverNeededParam
  Discrete-Time Integrator1 : DiscreteIntegrator  InitialConditionSource=external  SampleTime=-1  LimitOutput=on  UpperSaturationLimit=50  LowerSaturationLimit=-50  ICPrevOutput=DiscIntNeverNeededParam  ICPrevScaledInput=DiscIntNeverNeededParam
  Discrete-Time Integrator2 : DiscreteIntegrator  InitialConditionSource=external  InitialCondition=0.1  SampleTime=-1  LimitOutput=on  UpperSaturationLimit=50  LowerSaturationLimit=-50  ICPrevOutput=DiscIntNeverNeededParam  ICPrevScaledInput=DiscIntNeverNeededParam
  Divide : Product  Inputs=*/  OutMin=-50  OutMax=50
  Divide1 : Product  Inputs=*/  OutMin=-50  OutMax=50
  Divide2 : Product  Inputs=*/
  Index Vector{,1..13} (14 alike) : MultiPortSwitch  DataPortOrder=Zero-based contiguous  Inputs=1  zeroidx=on  SaturateOnIntegerOverflow=off  InputSameDT=off
  Mass (kg) : Constant  Value=222.26
  Product{,1..5} (6 alike) : Product
  Saturation : Saturate  UpperLimit=50  LowerLimit=-50
  Saturation1 : Saturate  UpperLimit=50  LowerLimit=-50
  Subtract : Sum  Inputs=+-
  fdrag (N) : Constant  Value=1.29
  front left{,1..3} (4 alike) : Constant  Value=0
  front right{,1..3} (4 alike) : Constant
  i_zz (Kgm^2) : Constant  Value=120
  l_f (m) : Constant  Value=0.77
  l_r (m) : Constant  Value=0.885
  max velocity : Constant  Value=50
  rear left : Constant  Value=2
  rear left1 : Constant  Value=2
  rear left2 : Constant  Value=2
  rear right : Constant  Value=3
  rear right1 : Constant  Value=3
  rear right2 : Constant  Value=3
  rear track (m) : Constant  Value=1.3208
  f_bx : ArgIn  DisableCoverage=on  PortDimensions=4  ArgumentName=f_bx
  f_by : ArgIn  Port=2  PortDimensions=4  ArgumentName=f_by
  f_bxroll : ArgIn  Port=3  PortDimensions=4  ArgumentName=f_bxroll
  f_byroll : ArgIn  Port=4  PortDimensions=2  ArgumentName=f_byroll
  v_x : ArgOut  DisableCoverage=on  OutMin=[-35]  OutMax=[35]  ArgumentName=v_x
  v_y : ArgOut  Port=2  OutMin=[-35]  OutMax=[35]  ArgumentName=v_y
  a_x : ArgOut  Port=3  OutMin=[-35]  OutMax=[35]  ArgumentName=a_x
  a_y : ArgOut  Port=4  OutMin=[-35]  OutMax=[35]  ArgumentName=a_y
  yaw_rate : ArgOut  Port=5  ArgumentName=yaw_rate
  yaw_accel : ArgOut  Port=6  ArgumentName=yaw_accel
  wires:
  fdrag (N)/1 -> Add1/6
  Add/1 -> Add1/5
  Index Vector/1 -> Add4/1, Add1/1
  Index Vector1/1 -> Add4/2, Add1/2
  Index Vector2/1 -> Add4/3, Add1/3
  Index Vector3/1 -> Add4/4, Add1/4
  Index Vector8/1 -> Add/1
  Index Vector9/1 -> Add/2
  Index Vector10/1 -> Add/3
  Index Vector11/1 -> Add/4
  Add1/1 -> Divide/1
  Mass (kg)/1 -> Divide1/2, Divide/2
  Divide/1 -> Saturation/1
  Index Vector4/1 -> Add5/1, Add2/1
  Index Vector5/1 -> Add5/2, Add2/2
  Index Vector6/1 -> Add2/3, Add6/1
  Index Vector7/1 -> Add2/4, Add6/2
  Index Vector12/1 -> Add3/1
  Index Vector13/1 -> Add3/2
  Add2/1 -> Subtract/1
  Add3/1 -> Subtract/2
  Subtract/1 -> Divide1/1
  Add4/1 -> Product/1
  rear track (m)/1 -> Product/2
  Add5/1 -> Product1/1
  l_f (m)/1 -> Product1/2
  Add6/1 -> Product2/1
  l_r (m)/1 -> Product2/2
  Product/1 -> Add7/1
  Product1/1 -> Add7/2
  Product2/1 -> Add7/3
  Add7/1 -> Divide2/1
  i_zz (Kgm^2)/1 -> Divide2/2
  Divide2/1 -> yaw_accel/1, Discrete-Time Integrator2/1, Product5/1
  f_bx/1 -> Index Vector3/2, Index Vector2/2, Index Vector1/2, Index Vector/2
  front right/1 -> Index Vector1/1
  rear left/1 -> Index Vector2/1
  rear right/1 -> Index Vector3/1
  f_by/1 -> Index Vector7/2, Index Vector6/2, Index Vector5/2, Index Vector4/2
  front left1/1 -> Index Vector4/1
  front right1/1 -> Index Vector5/1
  rear left1/1 -> Index Vector6/1
  rear right1/1 -> Index Vector7/1
  f_bxroll/1 -> Index Vector11/2, Index Vector10/2, Index Vector9/2, Index Vector8/2
  front left2/1 -> Index Vector8/1
  front right2/1 -> Index Vector9/1
  rear left2/1 -> Index Vector10/1
  rear right2/1 -> Index Vector11/1
  front right3/1 -> Index Vector13/1
  front left3/1 -> Index Vector12/1
  f_byroll/1 -> Index Vector13/2, Index Vector12/2
  front left/1 -> Index Vector/1
  Divide1/1 -> Saturation1/1
  Discrete-Time Integrator2/1 -> Data Store Write2/1, yaw_rate/1
  max velocity/1 -> ?
  Discrete-Time Integrator/1 -> v_y/1, Data Store Write1/1
  Discrete-Time Integrator1/1 -> Data Store Write/1, v_x/1
  Saturation/1 -> Discrete-Time Integrator1/1, a_x/1, Product3/1
  Saturation1/1 -> Data Store Write3/1, a_y/1, Product4/1, Discrete-Time Integrator/1
  Data Store Read/1 -> Product3/2
  Product3/1 -> Discrete-Time Integrator1/2
  Data Store Read1/1 -> Product4/2
  Product4/1 -> Discrete-Time Integrator/2
  Data Store Read2/1 -> Product5/2
  Product5/1 -> Discrete-Time Integrator2/2

== system torque_vectoring_sim/rolling resistance ==
  rollingresistance : TriggerPort  TriggerType=function-call  IsSimulinkFunction=on  FunctionName=rollingresistance  FunctionVisibility=scoped  VariantControl=(inherit)
  Index Vector{,1..3} (4 alike) : MultiPortSwitch  DataPortOrder=Zero-based contiguous  Inputs=1  zeroidx=on  SaturateOnIntegerOverflow=off  InputSameDT=off
  c_roll : Constant  Value=0.008
  front left : Constant  Value=0
  front right : Constant
  rear left : Constant  Value=2
  rear right : Constant  Value=3
  f_wx : ArgIn  DisableCoverage=on  ArgumentName=f_wx
  f_wy : ArgIn  Port=2  ArgumentName=f_wy
  ss_a : ArgIn  Port=3  ArgumentName=ss_a
  f_w : ArgOut  DisableCoverage=on  ArgumentName=f_w
  wires:
  f_wx/1 -> Index Vector3/2, Index Vector2/2, Index Vector1/2, Index Vector/2
  front left/1 -> Index Vector/1
  rear left/1 -> Index Vector2/1
  front right/1 -> Index Vector1/1
  rear right/1 -> Index Vector3/1

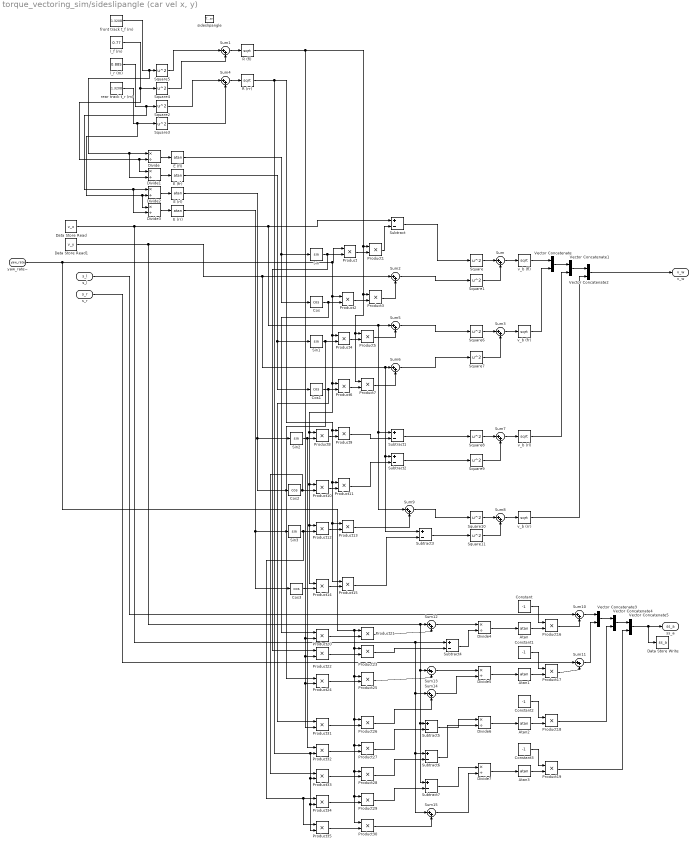
== system torque_vectoring_sim/sideslipangle (car vel x, y) ==
  sideslipangle : TriggerPort  TriggerType=function-call  IsSimulinkFunction=on  FunctionName=sideslipangle  FunctionVisibility=scoped  VariantControl=(inherit)
  Atan{,1..3} (4 alike) : Trigonometry  Operator=atan
  Constant{,1..3} (4 alike) : Constant  Value=-1
  Cos{,1..3} (4 alike) : Trigonometry  Operator=cos
  Data Store Read : DataStoreRead  DataStoreName=v_x  IndexOptions=Index vector (dialog)  Indices=1  OutputSizes=1
  Data Store Read1 : DataStoreRead  DataStoreName=v_y  IndexOptions=Index vector (dialog)  Indices=1  OutputSizes=1
  Data Store Write : DataStoreWrite  DataStoreName=ss_a  IndexOptions=Index vector (dialog)  Indices=1  OutputSizes=1
  Divide{,1..7} (8 alike) : Product  Inputs=*/
  E (fl) : Trigonometry  Operator=atan
  E (fr) : Trigonometry  Operator=atan
  E (rl) : Trigonometry  Operator=atan
  E (rr) : Trigonometry  Operator=atan
  Product{,1..35} (36 alike) : Product
  R (fl) : Sqrt
  R (rr) : Sqrt
  Sin{,1..3} (4 alike) : Trigonometry
  Square{,1..11} (12 alike) : Math  Operator=square
  Subtract{,1..7} (8 alike) : Sum  Inputs=+-
  Sum{,1..15} (16 alike) : Sum  Inputs=|++
  Vector Concatenate{,1..5} (6 alike) : Concatenate
  front track t_f (m) : Constant  Value=1.3208
  l_f (m) : Constant  Value=0.77
  l_r (m) : Constant  Value=0.885
  rear track t_r (m) : Constant  Value=1.3208
  v_b (fl) : Sqrt
  v_b (fr) : Sqrt
  v_b (rl) : Sqrt
  v_b (rr) : Sqrt
  yaw_rate~ : ArgIn  DisableCoverage=on  ArgumentName=yaw_rate
  s_l : ArgIn  Port=2  ArgumentName=s_l
  s_r : ArgIn  Port=3  ArgumentName=s_r
  v_w : ArgOut  DisableCoverage=on  PortDimensions=4  ArgumentName=v_w
  ss_a : ArgOut  Port=2  PortDimensions=4  ArgumentName=ss_a
  wires:
  Sum/1 -> v_b (fl)/1
  Square1/1 -> Sum/2
  Square/1 -> Sum/1
  front track t_f (m)/1 -> Divide1/2, Divide/1, Square5/1
  l_f (m)/1 -> Divide1/1, Divide/2, Square4/1
  rear track t_r (m)/1 -> Divide3/1, Divide2/2, Square3/1
  Sum1/1 -> R (fl)/1
  Sum4/1 -> R (rr)/1
  Square5/1 -> Sum1/1
  Square4/1 -> Sum1/2
  Square3/1 -> Sum4/2
  Square2/1 -> Sum4/1
  Divide/1 -> E (fl)/1
  Divide1/1 -> E (fr)/1
  Divide2/1 -> E (rl)/1
  Divide3/1 -> E (rr)/1
  l_r (m)/1 -> Divide3/2, Divide2/1, Square2/1
  Sin/1 -> Product22/1, Product/2
  Product/1 -> Product1/2
  Product1/1 -> Subtract/2
  Subtract/1 -> Square/1
  E (fl)/1 -> Cos/1, Sin/1
  Cos/1 -> Product20/1, Product2/2
  Product2/1 -> Product3/2
  Product3/1 -> Sum2/2
  Sum2/1 -> Square1/1
  Sum3/1 -> v_b (fr)/1
  Square6/1 -> Sum3/1
  Square7/1 -> Sum3/2
  Product5/1 -> Sum5/2
  Product4/1 -> Product5/2
  Sin1/1 -> Product24/1, Product4/2
  Product6/1 -> Product7/2
  Cos1/1 -> Product31/1, Product6/2
  Product7/1 -> Sum6/2
  Sum5/1 -> Square6/1
  Sum6/1 -> Square7/1
  E (fr)/1 -> Cos1/1, Sin1/1
  Sum7/1 -> v_b (rl)/1
  Square9/1 -> Sum7/2
  Square8/1 -> Sum7/1
  Subtract2/1 -> Square9/1
  Subtract1/1 -> Square8/1
  Sin2/1 -> Product32/1, Product8/2
  Product8/1 -> Product9/2
  Product9/1 -> Subtract1/2
  Product10/1 -> Product11/2
  Product11/1 -> Subtract2/2
  R (rr)/1 -> Product35/2, Product34/2, Product33/2, Product32/2, Product15/1, Product13/1, Product11/1, Product9/1
  E (rl)/1 -> Cos2/1, Sin2/1
  Sum8/1 -> v_b (rr)/1
  Square10/1 -> Sum8/1
  Square11/1 -> Sum8/2
  Subtract3/1 -> Square11/1
  Sum9/1 -> Square10/1
  E (rr)/1 -> Cos3/1, Sin3/1
  Product12/1 -> Product13/2
  Product13/1 -> Sum9/2
  Cos3/1 -> Product14/2
  Product14/1 -> Product15/2
  Product15/1 -> Subtract3/2
  v_b (fl)/1 -> Vector Concatenate/1
  v_b (fr)/1 -> Vector Concatenate/2
  Vector Concatenate/1 -> Vector Concatenate1/1
  v_b (rl)/1 -> Vector Concatenate1/2
  Vector Concatenate1/1 -> Vector Concatenate2/1
  v_b (rr)/1 -> Vector Concatenate2/2
  Vector Concatenate2/1 -> v_w/1
  Constant/1 -> Product16/1
  Atan/1 -> Product16/2
  Constant1/1 -> Product17/1
  Atan1/1 -> Product17/2
  Constant2/1 -> Product18/1
  Atan2/1 -> Product18/2
  Constant3/1 -> Product19/1
  Atan3/1 -> Product19/2
  Product16/1 -> Sum10/2
  Product17/1 -> Sum11/2
  Divide4/1 -> Atan/1
  Divide5/1 -> Atan1/1
  Divide7/1 -> Atan3/1
  Divide6/1 -> Atan2/1
  Sum12/1 -> Divide4/1
  Subtract4/1 -> Divide4/2
  Sum13/1 -> Divide5/1
  Sum14/1 -> Divide5/2
  Subtract5/1 -> Divide6/1
  Subtract6/1 -> Divide6/2
  Subtract7/1 -> Divide7/1
  Sum15/1 -> Divide7/2
  Product20/1 -> Product21/2
  Product21/1 -> Sum12/2
  Product22/1 -> Product23/2
  Product23/1 -> Subtract4/2
  Product24/1 -> Product25/2
  Product25/1 -> Sum13/2
  Product26/1 -> Sum14/2
  Product27/1 -> Subtract5/2
  Product28/1 -> Subtract6/2
  Product29/1 -> Subtract7/2
  Product30/1 -> Sum15/2
  Product31/1 -> Product26/2
  Product32/1 -> Product27/2
  Product33/1 -> Product28/2
  Product34/1 -> Product29/2
  Product35/1 -> Product30/2
  R (fl)/1 -> Product31/2, Product24/2, Product22/2, Product20/2, Product7/1, Product5/1, Product3/1, Product1/1
  Cos2/1 -> Product10/2, Product33/1
  Sin3/1 -> Product35/1, Product34/1, Product12/2
  Sum10/1 -> Vector Concatenate3/1
  Sum11/1 -> Vector Concatenate3/2
  Vector Concatenate3/1 -> Vector Concatenate4/1
  Product18/1 -> Vector Concatenate4/2
  Vector Concatenate4/1 -> Vector Concatenate5/1
  Product19/1 -> Vector Concatenate5/2
  Vector Concatenate5/1 -> Data Store Write/1, ss_a/1
  yaw_rate~/1 -> Product30/1, Product29/1, Product28/1, Product27/1, Product26/1, Product25/1, Product23/1, Product21/1, Product14/1, Product12/1, Product10/1, Product8/1, Product6/1, Product4/1, Product2/1, Product/1
  s_l/1 -> Sum10/1
  s_r/1 -> Sum11/1
  Data Store Read/1 -> Sum15/1, Subtract6/1, Sum14/1, Subtract4/1, Sum9/1, Subtract1/1, Sum5/1, Subtract/1
  Data Store Read1/1 -> Subtract7/1, Subtract5/1, Sum13/1, Sum12/1, Subtract3/1, Subtract2/1, Sum6/1, Sum2/1

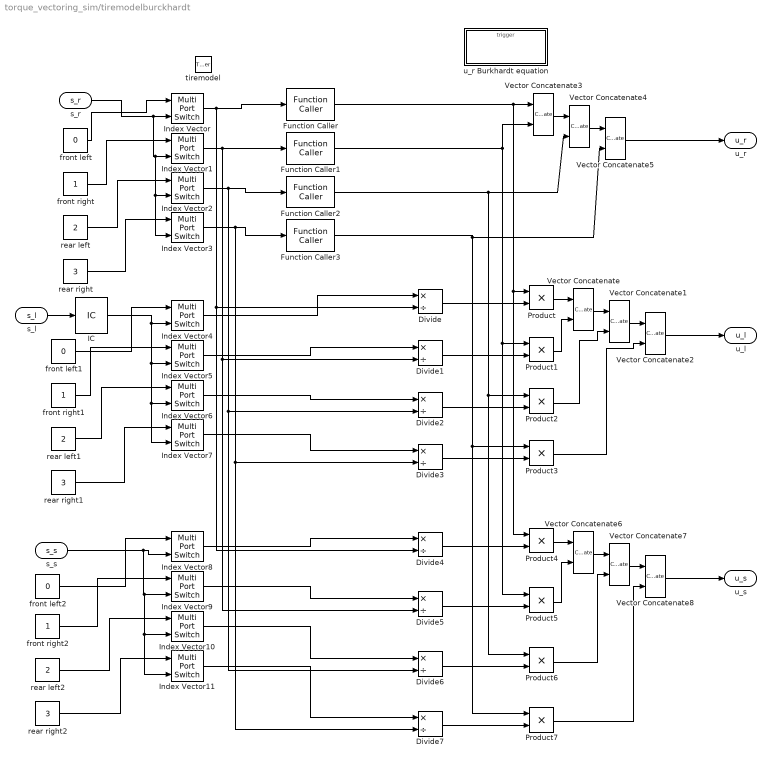
== system torque_vectoring_sim/tiremodelburckhardt ==
  tiremodel : TriggerPort  TriggerType=function-call  IsSimulinkFunction=on  FunctionName=tiremodel  FunctionVisibility=scoped  VariantControl=(inherit)
  Divide{,1..7} (8 alike) : Product  Inputs=*/
  Function Caller{,1..3} (4 alike) : FunctionCaller  FunctionPrototype=ur = burk(sr)  InputArgumentSpecifications=<Enter example>  OutputArgumentSpecifications=<Enter example>
  IC : InitialCondition  Value=[1, 1, 1, 1]
  Index Vector{,1..11} (12 alike) : MultiPortSwitch  DataPortOrder=Zero-based contiguous  Inputs=1  zeroidx=on  SaturateOnIntegerOverflow=off  InputSameDT=off
  Product{,1..7} (8 alike) : Product
  Vector Concatenate{,1..8} (9 alike) : Concatenate
  front left : Constant  Value=0
  front left1 : Constant  Value=0
  front left2 : Constant  Value=0
  front right : Constant
  front right1 : Constant
  front right2 : Constant
  rear left : Constant  Value=2
  rear left1 : Constant  Value=2
  rear left2 : Constant  Value=2
  rear right : Constant  Value=3
  rear right1 : Constant  Value=3
  rear right2 : Constant  Value=3
  u_r Burkhardt equation : Subsystem  TreatAsAtomicUnit=on
  s_r : ArgIn  DisableCoverage=on  PortDimensions=4  ArgumentName=s_r
  s_l : ArgIn  Port=2  PortDimensions=4  ArgumentName=s_l
  s_s : ArgIn  Port=3  PortDimensions=4  ArgumentName=s_s
  u_r : ArgOut  DisableCoverage=on  PortDimensions=4  ArgumentName=u_r
  u_l : ArgOut  Port=2  PortDimensions=4  ArgumentName=u_l
  u_s : ArgOut  Port=3  PortDimensions=4  ArgumentName=u_s
  wires:
  front right2/1 -> Index Vector9/1
  front left2/1 -> Index Vector8/1
  rear right2/1 -> Index Vector11/1
  rear left2/1 -> Index Vector10/1
  Index Vector/1 -> Divide4/2, Divide/2, Function Caller/1
  Index Vector1/1 -> Divide5/2, Divide1/2, Function Caller1/1
  Index Vector2/1 -> Divide6/2, Divide2/2, Function Caller2/1
  Index Vector3/1 -> Divide7/2, Divide3/2, Function Caller3/1
  Divide/1 -> Product/2
  Function Caller/1 -> Vector Concatenate3/1, Product4/1, Product/1
  Function Caller1/1 -> Vector Concatenate3/2, Product5/1, Product1/1
  Divide1/1 -> Product1/2
  Index Vector4/1 -> Divide/1
  Index Vector5/1 -> Divide1/1
  Function Caller2/1 -> Vector Concatenate4/2, Product6/1, Product2/1
  Divide2/1 -> Product2/2
  Index Vector6/1 -> Divide2/1
  Function Caller3/1 -> Vector Concatenate5/2, Product7/1, Product3/1
  Divide3/1 -> Product3/2
  Index Vector7/1 -> Divide3/1
  Divide4/1 -> Product4/2
  Divide6/1 -> Product6/2
  Divide5/1 -> Product5/2
  Divide7/1 -> Product7/2
  Index Vector8/1 -> Divide4/1
  Index Vector9/1 -> Divide5/1
  Index Vector10/1 -> Divide6/1
  Index Vector11/1 -> Divide7/1
  Product/1 -> Vector Concatenate/1
  Product1/1 -> Vector Concatenate/2
  Vector Concatenate/1 -> Vector Concatenate1/1
  Product2/1 -> Vector Concatenate1/2
  Vector Concatenate1/1 -> Vector Concatenate2/1
  Product3/1 -> Vector Concatenate2/2
  Vector Concatenate2/1 -> u_l/1
  Vector Concatenate4/1 -> Vector Concatenate5/1
  Vector Concatenate3/1 -> Vector Concatenate4/1
  Vector Concatenate5/1 -> u_r/1
  Vector Concatenate7/1 -> Vector Concatenate8/1
  Vector Concatenate6/1 -> Vector Concatenate7/1
  Product4/1 -> Vector Concatenate6/1
  Vector Concatenate8/1 -> u_s/1
  Product5/1 -> Vector Concatenate6/2
  Product6/1 -> Vector Concatenate7/2
  Product7/1 -> Vector Concatenate8/2
  s_r/1 -> Index Vector3/2, Index Vector2/2, Index Vector1/2, Index Vector/2
  front left/1 -> Index Vector/1
  front right/1 -> Index Vector1/1
  rear left/1 -> Index Vector2/1
  rear right/1 -> Index Vector3/1
  rear right1/1 -> Index Vector7/1
  rear left1/1 -> Index Vector6/1
  front right1/1 -> Index Vector5/1
  front left1/1 -> Index Vector4/1
  s_l/1 -> IC/1
  s_s/1 -> Index Vector11/2, Index Vector10/2, Index Vector9/2, Index Vector8/2
  IC/1 -> Index Vector7/2, Index Vector6/2, Index Vector5/2, Index Vector4/2

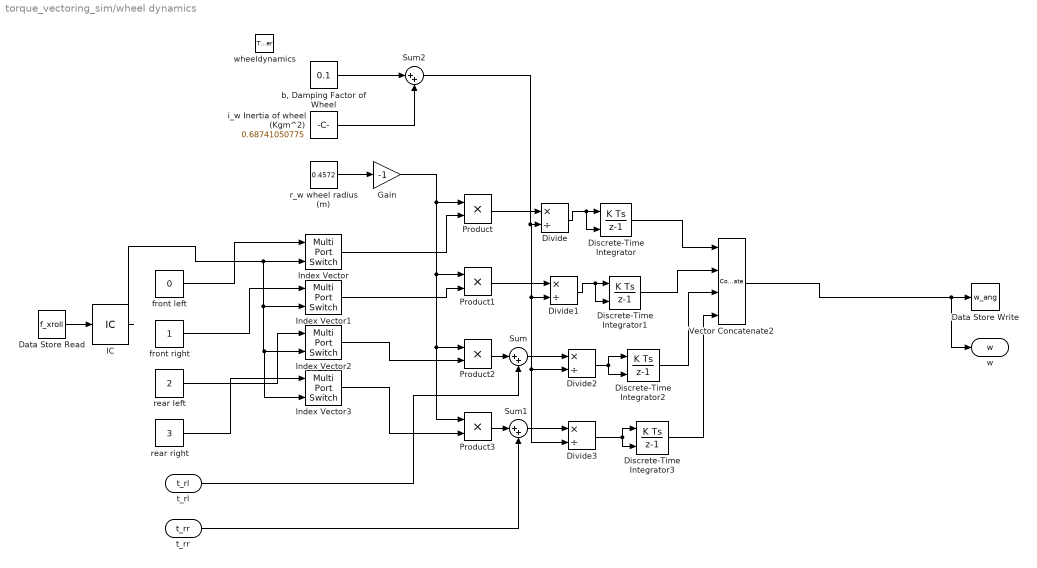
== system torque_vectoring_sim/wheel dynamics ==
  wheeldynamics : TriggerPort  TriggerType=function-call  IsSimulinkFunction=on  FunctionName=wheeldynamics  FunctionVisibility=scoped  VariantControl=(inherit)
  Data Store Read : DataStoreRead  DataStoreName=f_xroll  IndexOptions=Index vector (dialog)  Indices=1  OutputSizes=1
  Data Store Write : DataStoreWrite  DataStoreName=w_ang  IndexOptions=Index vector (dialog)  Indices=1  OutputSizes=1
  Discrete-Time Integrator{,1..3} (4 alike) : DiscreteIntegrator  InitialConditionSource=external  SampleTime=-1  ICPrevOutput=DiscIntNeverNeededParam  ICPrevScaledInput=DiscIntNeverNeededParam
  Divide{,1..3} (4 alike) : Product  Inputs=*/
  Gain : Gain  Gain=-1
  IC : InitialCondition  Value=[60, 60, 60, 60]
  Index Vector{,1..3} (4 alike) : MultiPortSwitch  DataPortOrder=Zero-based contiguous  Inputs=1  zeroidx=on  SaturateOnIntegerOverflow=off  InputSameDT=off
  Product{,1..3} (4 alike) : Product
  Sum : Sum  Inputs=|++
  Sum1 : Sum  Inputs=|++
  Sum2 : Sum  Inputs=|++
  Vector Concatenate2 : Concatenate  NumInputs=4
  "b, Damping Factor of Wheel" : Constant  Value=0.1
  front left : Constant  Value=0
  front right : Constant
  "i_w Inertia of wheel (Kgm^2) " : Constant  Value=0.68741050775
  r_w wheel radius (m) : Constant  Value=0.4572
  rear left : Constant  Value=2
  rear right : Constant  Value=3
  t_rr : ArgIn  DisableCoverage=on  ArgumentName=t_rr
  t_rl : ArgIn  Port=2  ArgumentName=t_rl
  w : ArgOut  DisableCoverage=on  PortDimensions=4  ArgumentName=w
  wires:
  IC/1 -> Index Vector1/2, Index Vector3/2, Index Vector2/2, Index Vector/2
  r_w wheel radius (m)/1 -> Gain/1
  Index Vector/1 -> Product/2
  Product/1 -> Divide/1
  Index Vector1/1 -> Product1/2
  Product1/1 -> Divide1/1
  Index Vector2/1 -> Product2/2
  Product2/1 -> Sum/1
  Sum/1 -> Divide2/1
  Gain/1 -> Product3/1, Product2/1, Product1/1, Product/1
  Index Vector3/1 -> Product3/2
  Product3/1 -> Sum1/1
  t_rl/1 -> Sum/2
  t_rr/1 -> Sum1/2
  Sum1/1 -> Divide3/1
  Discrete-Time Integrator/1 -> Vector Concatenate2/1
  Sum2/1 -> Divide3/2, Divide2/2, Divide1/2, Divide/2
  "b, Damping Factor of Wheel"/1 -> Sum2/1
  "i_w Inertia of wheel (Kgm^2) "/1 -> Sum2/2
  front right/1 -> Index Vector1/1
  front left/1 -> Index Vector/1
  rear left/1 -> Index Vector2/1
  rear right/1 -> Index Vector3/1
  Divide3/1 -> Discrete-Time Integrator3/2, Discrete-Time Integrator3/1
  Divide2/1 -> Discrete-Time Integrator2/2, Discrete-Time Integrator2/1
  Divide/1 -> Discrete-Time Integrator/2, Discrete-Time Integrator/1
  Divide1/1 -> Discrete-Time Integrator1/2, Discrete-Time Integrator1/1
  Discrete-Time Integrator1/1 -> Vector Concatenate2/2
  Discrete-Time Integrator2/1 -> Vector Concatenate2/3
  Discrete-Time Integrator3/1 -> Vector Concatenate2/4
  Vector Concatenate2/1 -> w/1, Data Store Write/1
  Data Store Read/1 -> IC/1
